simulink library "grid_element"  (R2025a)
settings: Solver=VariableStepAuto  StartTime=0.0  StopTime=10.0  RelTol=1e-3
undefined symbols (not defined in the file or in its folder): grid_clr, grid_num_sq_x, grid_opc, grid_x, grid_y, grid_z, hole_lx, hole_wx, SceneData, X, Y, Z
libraries: sm_lib x7, $bdroot x2
Description:
  | Copyright 2023-2025 The MathWorks, Inc.
settings Model: Creator=smiller  LastModifiedBy=smiller
settings RTWCC: GPUComputeCapability=3.5

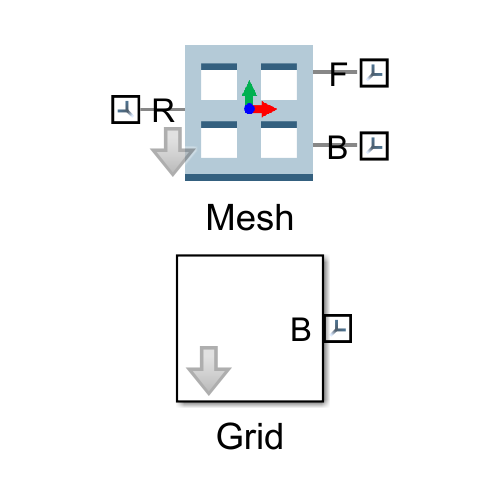
[thumbnail: Simulink's stored preview of the top-level diagram]
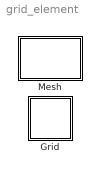
== system grid_element ==
  Grid : Subsystem  VariantControl=Grid  mask(Grid){grid_x=SceneData.Grid.length, grid_y=SceneData.Grid.width, grid_z=SceneData.Grid.depth, grid_line_width=SceneData.Grid.linewidth, grid_num_sq_x=SceneData.Grid.numsquaresx, grid_num_sq_y=SceneData.Grid.numsquaresy, grid_clr=SceneData.Grid.linecolor, plane_clr=SceneData.Grid.planecolor, grid_opc=1, plane_opc=1}
      mask prompts: grid_x "Length (m) (Global x)"; grid_y "Width (m) (Global y)"; grid_z "Depth (m) (Global z)"; grid_line_width "Line width (m)"; grid_num_sq_x "Number of squares in x"; grid_num_sq_y "Number of squares in y"; grid_clr "Line Color [RGB]"; plane_clr "Plane Color [RGB]"; grid_opc "Line Opacity (0-1)"; plane_opc "Plane Opacity (0-1)"
      mask help: Creates a grid for use in animations.
      mask init:
      | % Derived parameters - for two perpendicular grids with num_sq-by-1 holes
      | % **Note, not num_sq_x by num_sq_y holes - better render speed with
      | % separate meshes for x and y.
      | 
      | hole_lx = (grid_x-(grid_line_width*(grid_num_sq_x+1)))/grid_num_sq_x;
      | hole_wx = (grid_y-(grid_line_width*(1+1)))/1;
      | 
      | hole_ly = (grid_y-(grid_line_width*(grid_num_sq_y+1)))/grid_num_sq_y;
      | hole_wy = (grid_x-(grid_line_width*(1+1)))/1;
  Mesh : Subsystem  mask(Rectangular Mesh){mesh_lenx=grid_x, mesh_leny=grid_y, mesh_hx=hole_lx, mesh_hy=hole_wx, mesh_numhx=grid_num_sq_x, mesh_numhy=1, mesh_thickness=grid_z, mesh_rho=7000, mesh_color=grid_clr, mesh_opc=grid_opc}
      mask prompts: mesh_thickness "Thickness (m)"; mesh_rho "Density (kg/m^3)"; mesh_color "Color [RGB]"; mesh_opc "Opacity (0-1)"
      mask help: Rectangular mesh. Define outer dimensions, dimensions of holes, and thickness. R port is at the CG. Thickness defines the distance of the F frame from the B frame along the z-axis.
      mask init:
      | mesh_xsec = sm_extr_data_mesh(mesh_lenx, mesh_leny, mesh_numhx, mesh_numhy, mesh_hx, mesh_hy);
      mask DialogControl Control12 Prompt: Plot Profile
      mask DialogControl Control12 Callback:
      | v = get_param(gcb,'MaskWSVariables');
      | getMaskValue = containers.Map({v.Name}',{v.Value}');
      | evalin('base',...
      |     sprintf('Extr_Data_Mesh(%s,%s,%s,%s,%s,%s,''%s'');',...
      |     num2str(getMaskValue('mesh_lenx')),...
      |     num2str(getMaskValue('mesh_leny')),...
      |     num2str(getMaskValue('mesh_numhx')),...
      |     num2str(getMaskValue('mesh_numhy')),...
      |     num2str(getMaskValue('mesh_hx')),...
      |     num2str(getMaskValue('mesh_hy')),'plot'));
      mask DialogControl Control7 Prompt: X
      mask DialogControl Control8 Prompt: Y
      mask DialogControl Control9 Prompt: Mesh Length (m)
      mask DialogControl Control11 Prompt: Hole Length (m)
      mask DialogControl Control10 Prompt: Number of Holes
      mask Display: image('sm_parts_mesh_image.png');

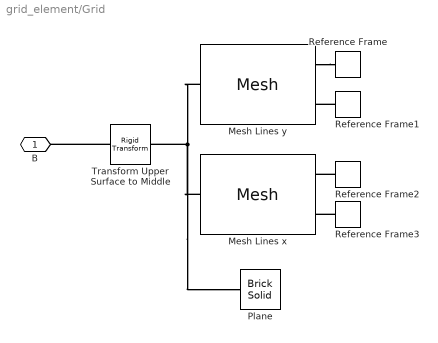
== system grid_element/Grid ==
  Mesh Lines x : $bdroot/Mesh  mesh_lenx=grid_x  mesh_leny=grid_y  mesh_hx=hole_wy  mesh_hy=hole_ly  mesh_numhx=1  mesh_numhy=grid_num_sq_y  mesh_thickness=grid_z  mesh_rho=7000  mesh_color=grid_clr  mesh_opc=grid_opc
  "Mesh Lines y " : $bdroot/Mesh  mesh_lenx=grid_x  mesh_leny=grid_y  mesh_hx=hole_lx  mesh_hy=hole_wx  mesh_numhx=grid_num_sq_x  mesh_numhy=1  mesh_thickness=grid_z  mesh_rho=7000  mesh_color=grid_clr  mesh_opc=grid_opc
  Plane : sm_lib/Body Elements/Brick Solid  BrickDimensions=[grid_x grid_y grid_z-0.01]  BrickDimensionsUnits=m  ExportEntireGeometry=off  InertiaType=CalculateFromGeometry  BasedOnType=Density  Density=1000  DensityUnits=kg/m^3  Mass=1  MassUnits=kg  CenterOfMass=[0 0 0]  CenterOfMassUnits=m  MomentsOfInertia=[1 1 1]  MomentsOfInertiaUnits=kg*m^2  ProductsOfInertia=[0 0 0]  ProductsOfInertiaUnits=kg*m^2  GraphicType=FromGeometry  MarkerShape=Sphere  MarkerSize=10  GraphicVisPropType=SimpleVisualProperties  GraphicDiffuseColor=plane_clr  GraphicOpacity=plane_opc  GraphicSpecularColor=[0.5 0.5 0.5 1.0]  GraphicAmbientColor=[0.15 0.15 0.15 1.0]  GraphicEmissiveColor=[0.0 0.0 0.0 1.0]  GraphicShininess=75  DoExposeReferenceFrame=on  SerializedFrames=<Frames/>
  Reference Frame{,1..3} (4 alike) : sm_lib/Frames and Transforms/Reference Frame
  Transform Upper Surface to Middle : sm_lib/Frames and Transforms/Rigid Transform  RotationMethod=None  FollAlignAxisA=+X  BaseAlignAxisA=+Y  FollAlignAxisB=+Y  BaseAlignAxisB=+Z  RotationStandardAxis=+Z  RotationAngle=0.0  RotationAngleUnits=deg  RotationArbitraryAxis=[0 0 1]  RotationSequenceAxes=FollowerAxes  RotationSequence=XYX  RotationSequenceAngles=[0 0 0]  RotationSequenceAnglesUnits=deg  RotationMatrix=[1 0 0; 0 1 0; 0 0 1]  Quaternion=[1 0 0 0]  TranslationMethod=StandardAxis  TranslationCartesianOffset=[0 0 0]  TranslationCartesianOffsetUnits=m  TranslationStandardAxis=+Z  TranslationStandardOffset=-grid_z/2  TranslationStandardOffsetUnits=m  TranslationROffset=0  TranslationROffsetUnits=m  TranslationThetaOffset=0  TranslationThetaOffsetUnits=deg  TranslationZOffset=0  TranslationZOffsetUnits=m
  B : PMIOPort  Side=Right
  connections:
  Reference Frame3/RConn1 -- Mesh Lines x/RConn2
  "Mesh Lines y "/LConn1 -- Transform Upper Surface to Middle/RConn1 -- Mesh Lines x/LConn1 -- Plane/RConn1
  "Mesh Lines y "/RConn1 -- Reference Frame/RConn1
  Reference Frame1/RConn1 -- "Mesh Lines y "/RConn2
  Reference Frame2/RConn1 -- Mesh Lines x/RConn1
  Transform Upper Surface to Middle/LConn1 -- B/RConn1

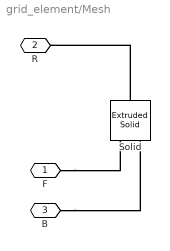
== system grid_element/Mesh ==
  Solid : sm_lib/Body Elements/Extruded Solid  ExtrusionType=General  PolygonNumSides=3  PolygonOuterRadius=1  PolygonOuterRadiusUnits=m  ExportEntireGeometry=off  ExtrusionCrossSection=mesh_xsec  ExtrusionCrossSectionUnits=m  ExportConvexHullGeometry=off  ExtrusionLength=mesh_thickness  ExtrusionLengthUnits=m  InertiaType=CalculateFromGeometry  BasedOnType=Density  Density=mesh_rho  DensityUnits=kg/(m^3)  Mass=1  MassUnits=kg  CenterOfMass=[0 0 0]  CenterOfMassUnits=m  MomentsOfInertia=[1 1 1]  MomentsOfInertiaUnits=kg*m^2  ProductsOfInertia=[0 0 0]  ProductsOfInertiaUnits=kg*m^2  GraphicType=FromGeometry  MarkerShape=Sphere  MarkerSize=10  GraphicVisPropType=AdvancedVisualProperties  GraphicDiffuseColor=mesh_color  GraphicOpacity=mesh_opc  GraphicSpecularColor=[0.5 0.5 0.5 1.0]  GraphicAmbientColor=[0.15 0.15 0.15 1.0]  GraphicEmissiveColor=[mesh_color 1.0]  GraphicShininess=75  DoExposeReferenceFrame=on  SerializedFrames=<Frames><Frame><Id>Frame1</Id><Value><Name>F</Name><Origin><Source>GeometricFeature</Source><FeatureName>top surface</FeatureName></Origin><PrimaryAxis><DefinedDirection>+Z</DefinedDirection><Source>ReferenceFrame</Source><SourceDirection>+Z</SourceDirection><FeatureName></FeatureName></PrimaryAxis><SecondaryAxis><DefinedDirection>+X</DefinedDirection><Source>ReferenceFrame</Source><SourceDirection>+X</SourceDirection><FeatureName></FeatureName></SecondaryAxis></Value></Frame><Frame><Id>Frame2</Id><Value><Name>B</Name><Origin><Source>GeometricFeature</Source><FeatureName>bottom surface</FeatureName></Origin><PrimaryAxis><DefinedDirection>+Z</DefinedDirection><Source>ReferenceFrame</Source><SourceDirection>+Z</SourceDirection><FeatureName></FeatureName></PrimaryAxis><SecondaryAxis><DefinedDirection>+X</DefinedDirection><Source>ReferenceFrame</Source><SourceDirection>+X</SourceDirection><FeatureName></FeatureName></SecondaryAxis></Value></Frame></Frames>
  F : PMIOPort  Side=Right
  R : PMIOPort  Port=2  Side=Left
  B : PMIOPort  Port=3  Side=Right
  connections:
  B/RConn1 -- Solid/LConn2
  F/RConn1 -- Solid/LConn1
  Solid/RConn1 -- R/RConn1
